simulink model "FSC"  (R2024b)
settings: Solver=FixedStepAuto  StartTime=0.0  StopTime=inf  FixedStep=0.001  RelTol=1e-3  EnableMultiTasking=on
libraries: px4Sensorslib x5, px4Peripheralslib x1
settings Model: SimulationMode=external  ExtModeTrigDuration=10  Creator=ArriGE66  LastModifiedBy=xippa
settings SolverCC: PositivePriorityOrder=on
settings OptimizationCC: EnhancedBackFolding=on  PassReuseOutputArgsAs=Individual arguments  ZeroExternalMemoryAtStartup=off  ZeroInternalMemoryAtStartup=off  MaxStackSize=64  OptimizeBlockOrder=speed  DifferentSizesBufferReuse=on  OptimizationCustomize=off  EfficientTunableParamExpr=on
settings DebuggingCC: ParameterTunabilityLossMsg=error
settings HardwareCC: ProdBitPerPointer=32  ProdBitPerSizeT=32  ProdBitPerPtrDiffT=32  ProdLargestAtomicInteger=Long  ProdLargestAtomicFloat=Double  ProdWordSize=32  ProdLongLongMode=on  ProdHWDeviceType=ARM Compatible->ARM Cortex
settings SFSimCC: MATLABDynamicMemAlloc=off  SimTargetLang=C++
settings RTWCC: Description=Embedded Coder  SystemTargetFile=ert.tlc  HardwareBoard=PX4 Cube Orange  TemplateMakefile=ert_default_tmf  Toolchain=GNU Tools for PX4 Autopilots  TargetLang=C++  GPUComputeCapability=3.5
settings CodeAppCC: ForceParamTrailComments=on  IgnoreCustomStorageClasses=off  OperatorAnnotations=on  SimulinkDataObjDesc=on  SFDataObjDesc=on  InsertBlockDesc=on
settings ERTTargetCC: SupportVariableSizeSignals=on  ExtMode=on  ExtModeTransport=3  ExtModeStaticAlloc=on  ExtModeStaticAllocSize=1024  ExtModeMexFile=ext_xcp  ExtModeMexArgs=1 COM10 3000000  ExtModeIntrfLevel=Level2 - Open  InlinedParameterPlacement=Hierarchical  DynamicArrayContainerType=coder::array

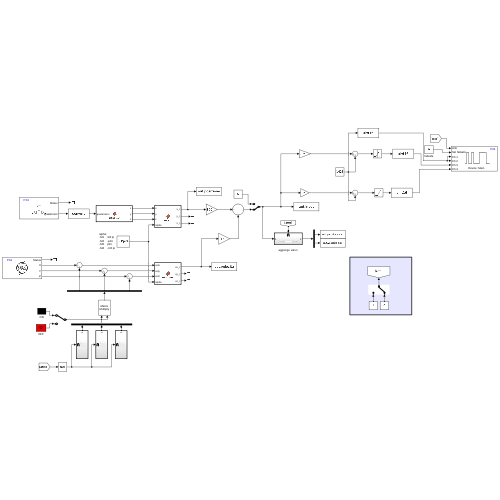
[thumbnail: Simulink's stored preview of the top-level diagram]
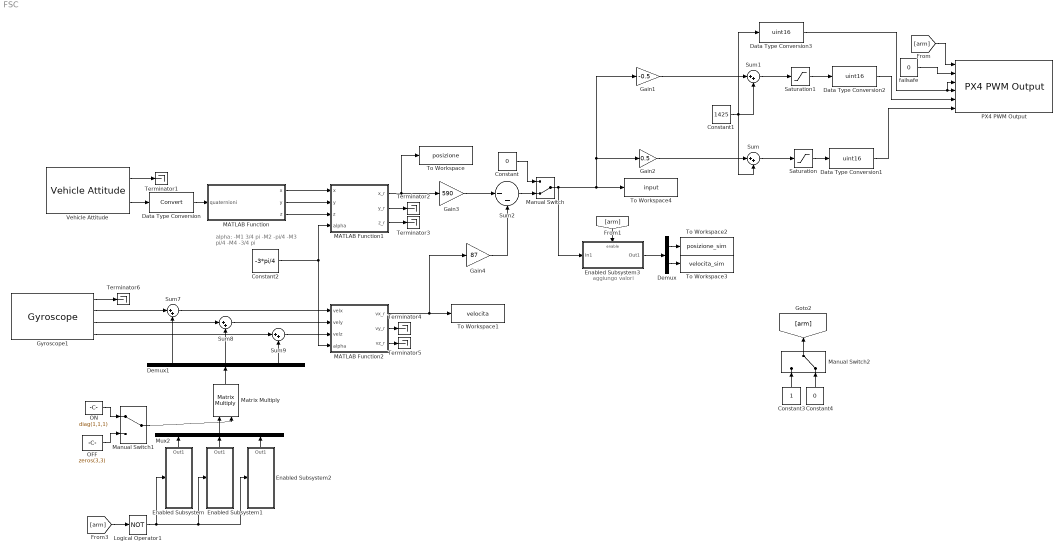
== system FSC ==
  note: aggiungo valori
  note: alpha:
      | -M1    3/4 pi
      | -M2    -pi/4
      | -M3    pi/4
      | -M4    -3/4 pi
  Constant : Constant  Value=0
  Constant1 : Constant  Value=1425  SampleTime=0.01
  Constant2 : Constant  Value=-3*pi/4  SampleTime=0.01
  Constant3 : Constant
  Constant4 : Constant  Value=0
  Data Type Conversion : DataTypeConversion  SaturateOnIntegerOverflow=off  RndMeth=Floor
  Data Type Conversion1 : DataTypeConversion  OutDataTypeStr=uint16  SaturateOnIntegerOverflow=off  RndMeth=Floor
  Data Type Conversion2 : DataTypeConversion  OutDataTypeStr=uint16  SaturateOnIntegerOverflow=off  RndMeth=Floor
  Data Type Conversion3 : DataTypeConversion  OutDataTypeStr=uint16  SaturateOnIntegerOverflow=off  RndMeth=Floor
  Demux : Demux  Outputs=2
  Demux1 : Demux  Outputs=3
  Enabled Subsystem : Subsystem  TreatAsAtomicUnit=on
  Enabled Subsystem1 : Subsystem  TreatAsAtomicUnit=on
  Enabled Subsystem2 : Subsystem  TreatAsAtomicUnit=on
  Enabled Subsystem3 : Subsystem  TreatAsAtomicUnit=on
  Gain1 : Gain  Gain=-0.5
  Gain2 : Gain  Gain=0.5
  Gain3 : Gain  Gain=590
  Gain4 : Gain  Gain=87
  Gyroscope1 : px4Sensorslib/Gyroscope  uorbTimeStamp=off  BlockingMode=off  BlockTimeout=1e-3  sampleTime=0.01
  Logical Operator1 : Logic  Operator=NOT  AllPortsSameDT=off  OutDataTypeStr=boolean
  MATLAB Function : MATLAB Function  TreatAsAtomicUnit=on
  MATLAB Function1 : MATLAB Function  TreatAsAtomicUnit=on
  MATLAB Function2 : MATLAB Function  TreatAsAtomicUnit=on
  Manual Switch : ManualSwitch  CurrentSetting=0
  Manual Switch1 : ManualSwitch
  Manual Switch2 : ManualSwitch  CurrentSetting=0
  Matrix Multiply : Product  Multiplication=Matrix(*)
  Mux2 : Mux  Inputs=3
  OFF : Constant  Value=zeros(3,3)
  ON : Constant  Value=diag(1,1,1)
  PX4 PWM Output : px4Peripheralslib/PX4 PWM Output  pwmDevice=Main  pwmChannel1_=on  pwmChannel2_=on  pwmChannel3_=on  pwmChannel4_=on  pwmChannel5_=off  pwmChannel6_=off  pwmChannel7_=off  pwmChannel8_=off
  Saturation : Saturate  UpperLimit=1750  LowerLimit=1050
  Saturation1 : Saturate  UpperLimit=1750  LowerLimit=1050
  Sum{,1,7..9} (5 alike) : Sum  Inputs=|++
  Sum2 : Sum  Inputs=|--
  Terminator{1..6} (6 alike) : Terminator
  To Workspace : ToWorkspace  VariableName=posizione  SaveFormat=Timeseries  SampleTime=-1
  To Workspace1 : ToWorkspace  VariableName=velocita  SaveFormat=Timeseries  SampleTime=-1
  To Workspace2 : ToWorkspace  VariableName=posizione_sim  SaveFormat=Timeseries  SampleTime=-1
  To Workspace3 : ToWorkspace  VariableName=velocita_sim  SaveFormat=Timeseries  SampleTime=-1
  To Workspace4 : ToWorkspace  VariableName=input  SaveFormat=Timeseries  SampleTime=-1
  Vehicle Attitude : px4Sensorslib/Vehicle Attitude  rollRate=off  pitchRate=off  yawRate=off  quaternion=on  uorbTimeStamp=off  BlockingMode=off  BlockTimeout=0.001  sampleTime=0.01
  failsafe : Constant  Value=0  OutDataTypeStr=boolean  SampleTime=0.01
  wires:
  Gain1/1 -> Sum1/1
  Data Type Conversion2/1 -> PX4 PWM Output/5
  Sum/1 -> Saturation/1
  Gain2/1 -> Sum/1
  MATLAB Function/2(y) -> MATLAB Function1/2(y)
  MATLAB Function/1(x) -> MATLAB Function1/1(x)
  MATLAB Function/3(z) -> MATLAB Function1/3(z)
  Constant1/1 -> Data Type Conversion3/1, Sum1/2, Sum/2
  MATLAB Function1/1(x_r) -> To Workspace/1, Gain3/1
  Data Type Conversion1/1 -> PX4 PWM Output/6
  failsafe/1 -> PX4 PWM Output/2
  Sum1/1 -> Saturation1/1
  Vehicle Attitude/2 -> Data Type Conversion/1
  Data Type Conversion3/1 -> PX4 PWM Output/3, PX4 PWM Output/4
  Constant2/1 -> MATLAB Function1/4(alpha), MATLAB Function2/4(alpha)
  MATLAB Function2/1(vx_r) -> To Workspace1/1, Gain4/1
  Vehicle Attitude/1 -> Terminator1/1
  Gain3/1 -> Sum2/1
  Gain4/1 -> Sum2/2
  Saturation/1 -> Data Type Conversion1/1
  Saturation1/1 -> Data Type Conversion2/1
  MATLAB Function1/3(z_r) -> Terminator3/1
  MATLAB Function1/2(y_r) -> Terminator2/1
  MATLAB Function2/3(vz_r) -> Terminator5/1
  MATLAB Function2/2(vy_r) -> Terminator4/1
  Gyroscope1/4 -> Sum9/1
  Gyroscope1/3 -> Sum8/1
  Gyroscope1/1 -> Terminator6/1
  Gyroscope1/2 -> Sum7/1
  Sum7/1 -> MATLAB Function2/1(velx)
  Sum8/1 -> MATLAB Function2/2(vely)
  Sum9/1 -> MATLAB Function2/3(velz)
  Sum2/1 -> Manual Switch/2
  Manual Switch/1 -> Enabled Subsystem3/1(In1), To Workspace4/1, Gain2/1, Gain1/1
  Constant/1 -> Manual Switch/1
  Data Type Conversion/1 -> MATLAB Function/1(quaternioni)
  Mux2/1 -> Matrix Multiply/1
  ON/1 -> Manual Switch1/1
  Manual Switch1/1 -> Matrix Multiply/2
  Matrix Multiply/1 -> Demux1/1
  Logical Operator1/1 -> Enabled Subsystem2/Enable, Enabled Subsystem1/Enable, Enabled Subsystem/Enable
  Enabled Subsystem2/1(Out1) -> Mux2/3
  OFF/1 -> Manual Switch1/2
  Enabled Subsystem/1(Out1) -> Mux2/1
  [arm] -> Logical Operator1/1
  Enabled Subsystem1/1(Out1) -> Mux2/2
  Demux1/1 -> Sum7/2
  Demux1/2 -> Sum8/2
  Demux1/3 -> Sum9/2
  Constant3/1 -> Manual Switch2/1
  Manual Switch2/1 -> [arm]
  Constant4/1 -> Manual Switch2/2
  [arm] -> PX4 PWM Output/1
  [arm] -> Enabled Subsystem3/Enable
  Enabled Subsystem3/1(Out1) -> Demux/1
  Demux/1 -> To Workspace2/1
  Demux/2 -> To Workspace3/1

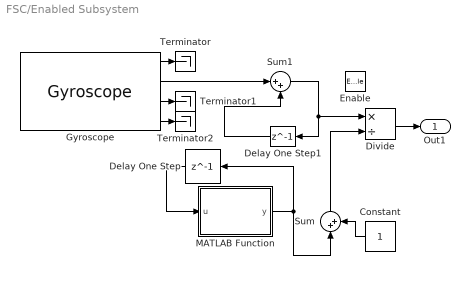
== system FSC/Enabled Subsystem ==
  Enable : EnablePort
  Constant : Constant
  Delay One Step : Delay  DelayLength=1
  Delay One Step1 : Delay  DelayLength=1
  Divide : Product  Inputs=*/
  Gyroscope : px4Sensorslib/Gyroscope  uorbTimeStamp=off  BlockingMode=off  BlockTimeout=1e-3  sampleTime=0.01
  MATLAB Function : MATLAB Function  TreatAsAtomicUnit=on
  Sum : Sum  Inputs=|++
  Sum1 : Sum  Inputs=|++
  Terminator : Terminator
  Terminator1 : Terminator
  Terminator2 : Terminator
  Out1 : Outport
  wires:
  Divide/1 -> Out1/1
  Sum1/1 -> Delay One Step1/1, Divide/1
  Sum/1 -> Divide/2
  Constant/1 -> Sum/2
  MATLAB Function/1(y) -> Delay One Step/1, Sum/1
  Delay One Step/1 -> MATLAB Function/1(u)
  Delay One Step1/1 -> Sum1/2
  Gyroscope/4 -> Terminator2/1
  Gyroscope/3 -> Terminator1/1
  Gyroscope/1 -> Terminator/1
  Gyroscope/2 -> Sum1/1

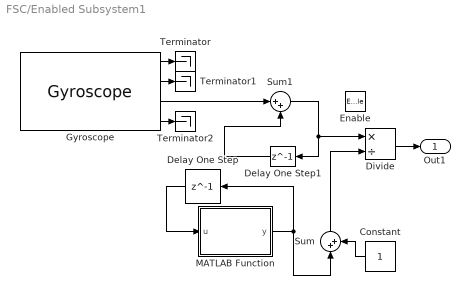
== system FSC/Enabled Subsystem1 ==
  Enable : EnablePort
  Constant : Constant
  Delay One Step : Delay  DelayLength=1
  Delay One Step1 : Delay  DelayLength=1
  Divide : Product  Inputs=*/
  Gyroscope : px4Sensorslib/Gyroscope  uorbTimeStamp=off  BlockingMode=off  BlockTimeout=1e-3  sampleTime=0.01
  MATLAB Function : MATLAB Function  TreatAsAtomicUnit=on
  Sum : Sum  Inputs=|++
  Sum1 : Sum  Inputs=|++
  Terminator : Terminator
  Terminator1 : Terminator
  Terminator2 : Terminator
  Out1 : Outport
  wires:
  Divide/1 -> Out1/1
  Sum1/1 -> Delay One Step1/1, Divide/1
  Sum/1 -> Divide/2
  Constant/1 -> Sum/2
  MATLAB Function/1(y) -> Delay One Step/1, Sum/1
  Delay One Step/1 -> MATLAB Function/1(u)
  Delay One Step1/1 -> Sum1/2
  Gyroscope/4 -> Terminator2/1
  Gyroscope/1 -> Terminator/1
  Gyroscope/3 -> Sum1/1
  Gyroscope/2 -> Terminator1/1

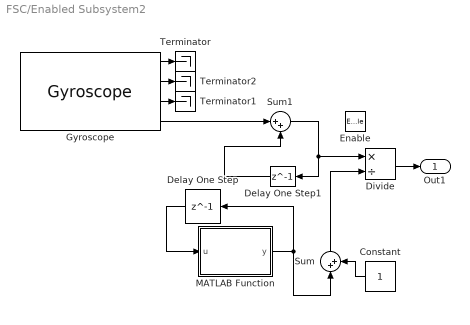
== system FSC/Enabled Subsystem2 ==
  Enable : EnablePort
  Constant : Constant
  Delay One Step : Delay  DelayLength=1
  Delay One Step1 : Delay  DelayLength=1
  Divide : Product  Inputs=*/
  Gyroscope : px4Sensorslib/Gyroscope  uorbTimeStamp=off  BlockingMode=off  BlockTimeout=1e-3  sampleTime=0.01
  MATLAB Function : MATLAB Function  TreatAsAtomicUnit=on
  Sum : Sum  Inputs=|++
  Sum1 : Sum  Inputs=|++
  Terminator : Terminator
  Terminator1 : Terminator
  Terminator2 : Terminator
  Out1 : Outport
  wires:
  Divide/1 -> Out1/1
  Sum1/1 -> Delay One Step1/1, Divide/1
  Sum/1 -> Divide/2
  Constant/1 -> Sum/2
  MATLAB Function/1(y) -> Delay One Step/1, Sum/1
  Delay One Step/1 -> MATLAB Function/1(u)
  Delay One Step1/1 -> Sum1/2
  Gyroscope/3 -> Terminator1/1
  Gyroscope/1 -> Terminator/1
  Gyroscope/4 -> Sum1/1
  Gyroscope/2 -> Terminator2/1

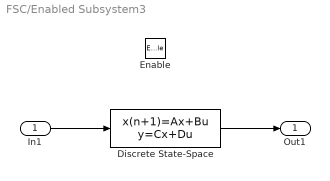
== system FSC/Enabled Subsystem3 ==
  In1 : Inport
  Enable : EnablePort
  Discrete State-Space : DiscreteStateSpace  SampleTime=-1
  Out1 : Outport
  wires:
  In1/1 -> Discrete State-Space/1
  Discrete State-Space/1 -> Out1/1

== matlab function FSC/MATLAB Function1 ==
  data: x input; y input; z input; x_r output; alpha input; y_r output; z_r output
function [x_r,y_r,z_r] = ruoto(x,y,z,alpha)
Global_POV = [x y z];
R_z = [cos(alpha), -sin(alpha), 0;
       sin(alpha), cos(alpha), 0;
       0, 0, 1];
LOCALPOV = Global_POV * R_z;
x_r = LOCALPOV(1);
y_r = LOCALPOV(2);
z_r = LOCALPOV(3);
end

== matlab function FSC/MATLAB Function ==
  data: x output; y output; quaternioni input; z output
function [x, y, z] = assetto(quaternioni)
    % Estrazione dei componenti del quaternione
    qw = quaternioni(1);
    qx = quaternioni(2);
    qy = quaternioni(3);
    qz = quaternioni(4);

    % Calcolo degli angoli di Eulero manualmente
    x = atan2(2*(qw*qx + qy*qz), 1 - 2*(qx^2 + qy^2)); % roll
    y = asin(2*(qw*qy - qz*qx));                          % Pitch
    z = atan2(2*(qw*qz + qx*qy), 1 - 2*(qy^2 + qz^2));   % yaw
end

== matlab function FSC/MATLAB Function2 ==
  data: velx input; vely input; velz input; vx_r output; alpha input; vy_r output; vz_r output
function [vx_r,vy_r,vz_r] = ruotovel(velx,vely,velz,alpha)
Global_POV = [velx vely velz];
R_z = [cos(alpha), -sin(alpha), 0;
       sin(alpha), cos(alpha), 0;
       0, 0, 1];
LOCALPOV = Global_POV * R_z;
vx_r = LOCALPOV(1);
vy_r = LOCALPOV(2);
vz_r = LOCALPOV(3);
end

== matlab function FSC/Enabled Subsystem/MATLAB Function ==
  data: u input; y output
function y = fcn(u)
y = u+1;

== matlab function FSC/Enabled Subsystem1/MATLAB Function ==
  data: u input; y output
function y = fcn(u)
y = u+1;

== matlab function FSC/Enabled Subsystem2/MATLAB Function ==
  data: u input; y output
function y = fcn(u)
y = u+1;
